simulink model "dc_motor_pid_simscape"  (R2026a)
settings: Solver=ode23t  StopTime=12  MaxStep=0.001  RelTol=1e-08  AbsTol=1e-10
model workspace (MAT data in the model file):
  Kb = 4.93696219862
  Kd = 1.84809830698
  Ki = 45.0448010417
  Kp = 17.9594547575
  Nf = 194.356054433
  Reference = 100
  TorqueTime = 1
  TorqueValue = 0
  VinValue = 12
  Vmax = 48
  Vmin = -48
  beta = 1
  gamma = 0
  p.Ra = 2
  p.La = 0.5
  p.Kt = 0.1
  p.Ke = 0.1
  p.Jm = 0.01
  p.Bm = 0.001
  p.JL = 0.02
  p.J = 0.03
  p.B = 0.001
  p.w_ref = 100
  p.Vmin = -48
  p.Vmax = 48
  p.beta = 1
  p.gamma = 0
  p.derivativeRatio = 20
  p.minimumFilterTime = 0.001
  p.ts_spec = 2
  p.os_spec = 5
  p.ess_spec = 0.2
  p.band = 0.02
  p.dt = 0.001
  p.RelTol = 1e-08
  p.AbsTol = 1e-10
  p.seed = 7
  p.Tsim = 5
  p.Tsim_ol = 30
  p.TL_step = 0.05
  p.TL_time = 1
  p.config.schemaVersion = 1
  p.config.physical.Ra = 2
  p.config.physical.La = 0.5
  p.config.physical.Kt = 0.1
  p.config.physical.Ke = 0.1
  p.config.physical.Jm = 0.01
  p.config.physical.Bm = 0.001
  p.config.physical.JL = 0.02
  p.config.control.reference = 100
  p.config.control.Vmin = -48
  p.config.control.Vmax = 48
  p.config.control.beta = 1
  p.config.control.gamma = 0
  p.config.control.derivativeRatio = 20
  p.config.control.minimumFilterTime = 0.001
  p.config.control.antiWindup = 'back-calculation'
  p.config.chosenTargets.settlingBand = 0.02
  p.config.chosenTargets.settlingTime = 2
  p.config.chosenTargets.overshootPercent = 5
  p.config.chosenTargets.steadyError = 0.2
  p.config.numerics.relativeTolerance = 1e-08
  p.config.numerics.absoluteTolerance = 1e-10
  p.config.numerics.outputStep = 0.001
  p.config.numerics.seed = 7
  p.config.assumptions = {'Bipolar +/-48 V is an engineering choice; the assignment specifies no voltage limit.'; 'Overshoot <=5% and steady error <=0.2 rad/s are chosen targets, not instructor-specified limits.'; 'The rigid load adds inertia only. Positive load torque opposes positive rotation.'}
  x0 = [0; 0]
libraries: fl_lib x7, nesl_utility x5, ee_lib x1, slpidlib x1
settings Model: Creator=ievge  LastModifiedBy=ievge

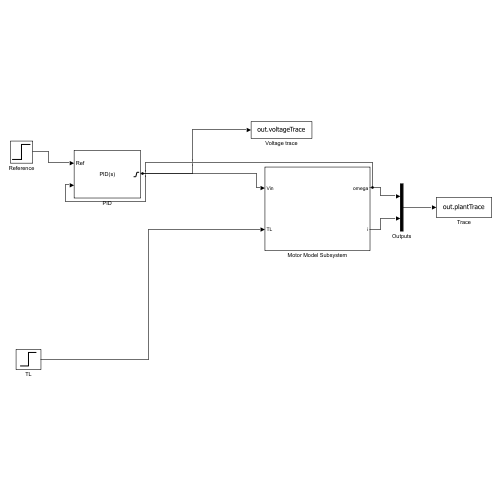
[thumbnail: Simulink's stored preview of the top-level diagram]
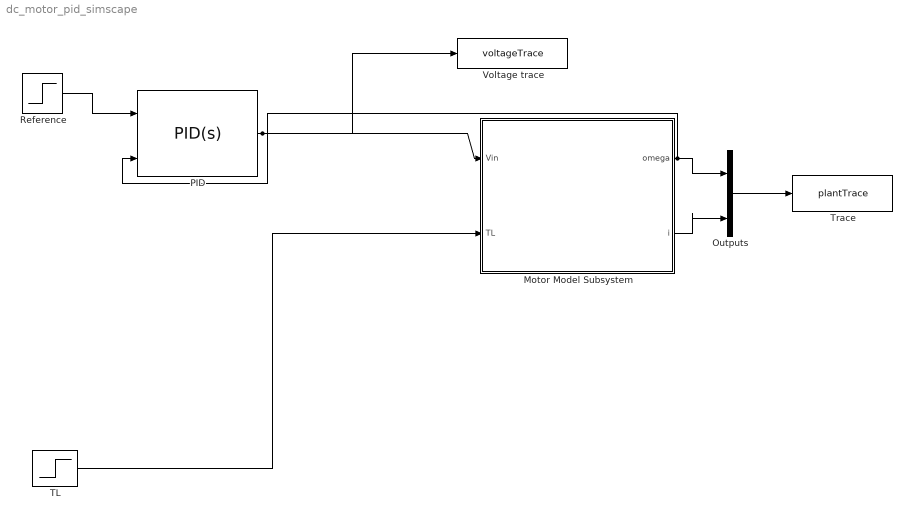
== system dc_motor_pid_simscape ==
  Motor Model Subsystem : Subsystem
  Outputs : Mux  Inputs=2
  PID : slpidlib/PID Controller (2DOF)  Controller=PID  Form=Parallel  TimeDomain=Continuous-time  UseExternalTs=off  SampleTime=-1  IntegratorMethod=Forward Euler  FilterMethod=Forward Euler  ControllerParametersSource=internal  P=Kp  I=Ki  UseKiTs=off  D=Kd  UseExternalDerivativeSource=off  N=Nf  UseFilter=on  b=beta  c=gamma  TunerSelectOption=Transfer Function Based (PID Tuner App)  InitialConditionSource=internal  InitialConditionForIntegrator=0  InitialConditionForFilter=0  DifferentiatorICPrevScaledInput=0  ExternalReset=none  TrackingMode=off  Kt=1  LimitOutput=on  SatLimitsSource=internal  UpperSaturationLimit=Vmax  LowerSaturationLimit=Vmin  LinearizeAsGain=on  AntiWindupMode=back-calculation  Kb=Kb  LimitIntegrator=off  UpperIntegratorSaturationLimit=inf  LowerIntegratorSaturationLimit=-inf  POutMin=[]  POutMax=[]  IOutMin=[]  IOutMax=[]  DOutMin=[]  DOutMax=[]  NOutMin=[]  NOutMax=[]  bOutMin=[]  bOutMax=[]  cOutMin=[]  cOutMax=[]  SumOutMin=[]  SumOutMax=[]  SaturationOutMin=[]  SaturationOutMax=[]  PParamMin=[]  PParamMax=[]  IParamMin=[]  IParamMax=[]  DParamMin=[]  DParamMax=[]  NParamMin=[]  NParamMax=[]  bParamMin=[]  bParamMax=[]  cParamMin=[]  cParamMax=[]  KbParamMin=[]  KbParamMax=[]  KtParamMin=[]  KtParamMax=[]  KbOutMin=[]  KbOutMax=[]  KtOutMin=[]  KtOutMax=[]  IntegratorOutMin=[]  IntegratorOutMax=[]  FilterOutMin=[]  FilterOutMax=[]  SumI1OutMin=[]  SumI1OutMax=[]  SumI2OutMin=[]  SumI2OutMax=[]  SumI3OutMin=[]  SumI3OutMax=[]  SumI4OutMin=[]  SumI4OutMax=[]  SumDOutMin=[]  SumDOutMax=[]  Sum1OutMin=[]  Sum1OutMax=[]  Sum2OutMin=[]  Sum2OutMax=[]  Sum3OutMin=[]  Sum3OutMax=[]  DifferentiatorOutMin=[]  DifferentiatorOutMax=[]  FilterDiffOutCoefMin=[]  FilterDiffOutCoefMax=[]  ReciprocalOutMin=[]  ReciprocalOutMax=[]  SumDenOutMin=[]  SumDenOutMax=[]  SumNumOutMin=[]  SumNumOutMax=[]  DivideOutMin=[]  DivideOutMax=[]  UdiffTsProdOutMin=[]  UdiffTsProdOutMax=[]  NTsProdOutMin=[]  NTsProdOutMax=[]  UintegralTsProdOutMin=[]  UintegralTsProdOutMax=[]  UngainTsProdOutMin=[]  UngainTsProdOutMax=[]  ClampingZeroOutDataTypeStr=Inherit: Inherit via back propagation  ClampingZeroOutMin=[]  ClampingZeroOutMax=[]  FilterDenConstantOutDataTypeStr=Inherit: Inherit via back propagation  FilterDenConstantOutMin=[]  FilterDenConstantOutMax=[]  PCopyOutDataTypeStr=Inherit: Inherit via back propagation  PCopyOutMin=[]  PCopyOutMax=[]  NCopyOutDataTypeStr=Inherit: Inherit via back propagation  NCopyOutMin=[]  NCopyOutMax=[]  IntegratorContinuousStateAttributes=''  IntegratorStateMustResolveToSignalObject=off  IntegratorRTWStateStorageClass=Auto  FilterContinuousStateAttributes=''  FilterStateMustResolveToSignalObject=off  FilterRTWStateStorageClass=Auto  ParallelPVariant=InternalParameters  IdealPVariant=Disabled  IVariant=InternalParameters  DVariant=InternalParameters  bVariant=InternalParameters  cVariant=InternalParameters  IntegratorVariant=Continuous  SatVariant=Enabled  AWVariant=BackCalculation  PCopyVariant=Disabled  TRVariant=Disabled  FdbkBlocksVariant=Forward  IdealPFdbkVariant=Disabled  SatFdbkVariant=Disabled  DerivativeFilterVariant=ContFilter  NVariant=InternalParameters  NCopyVariant=Disabled  FilterICVariant=InternalICsFilter  IntegratorICVariant=InternalICs  ExternalResetVariant=Disabled  TRSumVariant=Passthrough  SumFdbkVariant=Disabled  SumVariant=Sum_PID  TsampFilterVariant=InternalTs  TsampNgainVariant=Passthrough  TsampIntegralVariant=Disabled_SignalSpec  ExternalSaturationOutDataTypeStr=Inherit: Same as second input  DerivativeSourceVariant=ErrorSignal  PreIntVariant=InternalPreInt
  Reference : Step  Time=0  FinalValue=Reference  SampleTime=0
  TL : Step  Time=TorqueTime  FinalValue=TorqueValue  SampleTime=0
  Trace : ToWorkspace  VariableName=plantTrace  SaveFormat=Timeseries  SampleTime=-1
  Voltage trace : ToWorkspace  VariableName=voltageTrace  SaveFormat=Timeseries  SampleTime=-1
  wires:
  Outputs/1 -> Trace/1
  Reference/1 -> PID/1
  Motor Model Subsystem/1(omega) -> PID/2, Outputs/1
  PID/1 -> Motor Model Subsystem/1(Vin), Voltage trace/1
  TL/1 -> Motor Model Subsystem/2(TL)
  Motor Model Subsystem/2(i) -> Outputs/2

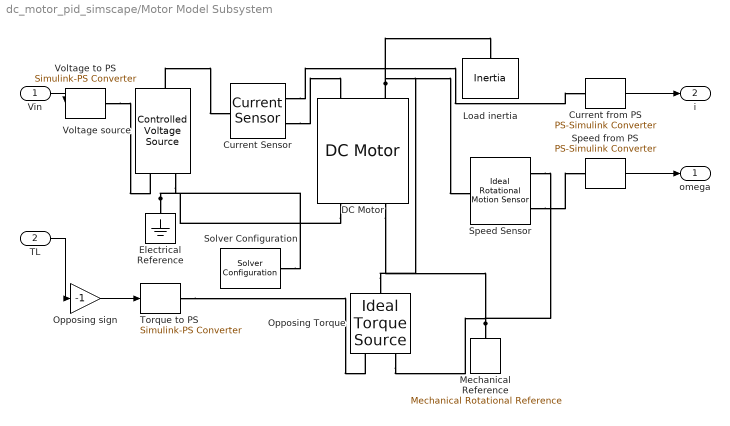
== system dc_motor_pid_simscape/Motor Model Subsystem ==
  Vin : Inport
  TL : Inport  Port=2
  Current Sensor : fl_lib/Electrical/Electrical Sensors/Current Sensor
  Current from PS : nesl_utility/PS-Simulink Converter  PhysicalDomain=network_engine_domain  SubClassName=ps_output  LeftPortType=input  RightPortType=output  PseudoPeriodic=off  Frequencies=[]  VectorFormat=inherit  Unit=A  AffineConversion=off
  DC Motor : ee_lib/Electromechanical/Brushed Motors/DC Motor  field_option=ee.enum.field_option.pm  Rf=100 Ohm  Lf=1 H  Laf=0.15 H  If0=0 A  parameterization=ee.enum.dcparam_option.circuit_param  Ra=p.Ra Ohm  La=p.La H  emf_or_torque=ee.enum.emf_or_torque.ki  Kv=0.072e-3 V/rpm  Ki=p.Kt N*m/A  T_stall=0.24e-3 N*m  w_max=19100 rpm  w_rated=15000 rpm  P_rated=0.08 W  V_rated=1.5 V  lam_param=ee.enum.lam_param.damping  i_noload=0 A  V_i_noload=1.5 V  J=p.Jm kg*m^2  lam=p.Bm N*m*s/rad  speed0=x0(2) rad/s  alpha=3.93e-3 1/K  Tmeas=25 degC  thermal_mass=100 J/K  initial_temperature=25 degC
  Electrical Reference : fl_lib/Electrical/Electrical Elements/Electrical Reference
  Load inertia : fl_lib/Mechanical/Rotational Elements/Inertia  inertia=p.JL kg*m^2  num_ports=foundation.enum.numPorts2.one  w_specify=off  w_priority=High  w=0 rad/s  w_nominal_specify=off  w_nominal_value=1  w_nominal_unit=rad/s  t_specify=off  t_priority=None  t=0 N*m  t_nominal_specify=off  t_nominal_value=1  t_nominal_unit=N*m
  Mechanical Reference : fl_lib/Mechanical/Rotational Elements/Mechanical Rotational Reference
  Opposing Torque : fl_lib/Mechanical/Mechanical Sources/Ideal Torque Source
  Opposing sign : Gain  Gain=-1
  Solver Configuration : nesl_utility/Solver Configuration  PhysicalDomain=network_engine_domain  SubClassName=solver  LeftPortType=input  RightPortType=generic  Tones=[]  Harmonics=[]  SimulateNoise=off  Profile=off  UseLocalSampling=off  EnableSwitchedLinearOptims=on  FrequencyDomain=off  UseCCode=off  RelTol=0.001  AbsTol=0.001  MinStep=1e-09  ToWorkspace=off  RevertToSquareIcSolve=off  NumHomotopyIterations=100  PhasorMode=off  PhasorModeNumHarmonics=1  ConsistencySolver=NEWTON_XTOL_AFTER_FTOL  CanonicalOrdering=CANONICAL  OptimizeIntermediates=OPTIMIZED  IndexReductionMethod=DerivativeReplacement  DoDC=off  ResidualTolerance=1e-09  ConsistencyTolSource=GLOBAL  ConsistencyAbsTol=0.001  ConsistencyRelTol=0.001  ConsistencyTolFactor=0.001  UseLocalSolver=off  LocalSolverChoice=NE_BACKWARD_EULER_ADVANCER  ResolveIndetEquations=on  FunctionEvalNumThread=1  LocalSolverSampleTime=0.001  DoFixedCost=off  MaxNonlinIter=3  MaxModeIter=2  ComputeImpulses=off  ImpulseIterations=2  LinearAlgebra=auto  LinearAlgebraNumThread=0  EquationFormulation=NE_TIME_EF  DelaysMemoryBudget=1024  AutomaticFiltering=on  FilteringTimeConstant=0.001  PartitionStorageMethod=AS_NEEDED  PartitionMemoryBudget=1024  PartitionMethod=ROBUST  MultibodyUseLocalSolver=off  MultibodyLocalSolverChoice=ODE1  MultibodyLocalSolverSampleTime=0.001
  Speed Sensor : fl_lib/Mechanical/Mechanical Sensors/Ideal Rotational Motion Sensor  reference=foundation.enum.MeasurementReference.difference  acceleration_port=false  velocity_port=true  position_port=false  wrap_angle=false  offset=0 rad
  Speed from PS : nesl_utility/PS-Simulink Converter  PhysicalDomain=network_engine_domain  SubClassName=ps_output  LeftPortType=input  RightPortType=output  PseudoPeriodic=off  Frequencies=[]  VectorFormat=inherit  Unit=rad/s  AffineConversion=off
  Torque to PS : nesl_utility/Simulink-PS Converter  PhysicalDomain=network_engine_domain  SubClassName=ps_input  LeftPortType=input  RightPortType=output  PseudoPeriodic=off  Frequencies=[]  NoiseDistribution=none  NoiseParameters=[]  Unit=N*m  AffineConversion=off  FilteringAndDerivatives=provide  SimscapeFilterOrder=1  InputFilterTimeConstant=0.001  UdotUserProvided=0
  Voltage source : fl_lib/Electrical/Electrical Sources/Controlled Voltage Source
  Voltage to PS : nesl_utility/Simulink-PS Converter  PhysicalDomain=network_engine_domain  SubClassName=ps_input  LeftPortType=input  RightPortType=output  PseudoPeriodic=off  Frequencies=[]  NoiseDistribution=none  NoiseParameters=[]  Unit=V  AffineConversion=off  FilteringAndDerivatives=provide  SimscapeFilterOrder=1  InputFilterTimeConstant=0.001  UdotUserProvided=0
  omega : Outport
  i : Outport  Port=2
  wires:
  Current from PS/1 -> i/1
  Speed from PS/1 -> omega/1
  Opposing sign/1 -> Torque to PS/1
  TL/1 -> Opposing sign/1
  Vin/1 -> Voltage to PS/1
  connections:
  Speed Sensor/RConn2 -- Speed from PS/LConn1
  Torque to PS/RConn1 -- Opposing Torque/RConn1
  Opposing Torque/RConn2 -- Mechanical Reference/LConn1 -- Speed Sensor/RConn1 -- DC Motor/RConn2
  Opposing Torque/LConn1 -- Speed Sensor/LConn1 -- Load inertia/LConn1 -- DC Motor/LConn2
  Current Sensor/RConn1 -- Current from PS/LConn1
  Solver Configuration/RConn1 -- Electrical Reference/LConn1 -- Voltage source/RConn2 -- DC Motor/RConn1
  Current Sensor/RConn2 -- DC Motor/LConn1
  Voltage source/LConn1 -- Current Sensor/LConn1
  Voltage to PS/RConn1 -- Voltage source/RConn1
